simulink model "UorbRead"  (R2026a)
settings: Solver=FixedStepAuto  StopTime=inf  EnableMultiTasking=on
libraries: px4Peripheralslib x1, px4uORBlib x1
settings Model: ExtModeTrigDuration=10  Creator=Carlos Fabian  LastModifiedBy=Carlos Fabian
settings SolverCC: PositivePriorityOrder=on
settings HardwareCC: ProdLargestAtomicInteger=Long  ProdLargestAtomicFloat=Double  ProdHWDeviceType=ARM Compatible->ARM Cortex
settings SFSimCC: SimTargetLang=C++
settings RTWCC: SystemTargetFile=ert.tlc  HardwareBoard=PX4 Host Target  TLCOptions="-aInlineSetEventsForThisBaseRateFcn=TLC_FALSE -aSuppressMultiTaskScheduler=TLC_FALSE  -aRateBasedStepFcn=0"  Toolchain=GNU Tools for PX4 Autopilots  PortableWordSizes=on  TargetLang=C++  Description=Embedded Coder
settings ERTTargetCC: ExtModeTransport=2.0

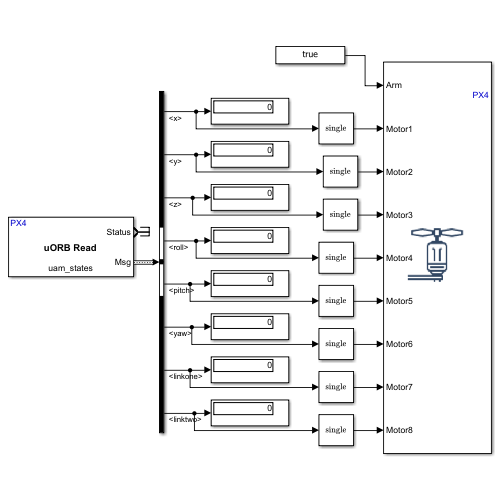
[thumbnail: Simulink's stored preview of the top-level diagram]
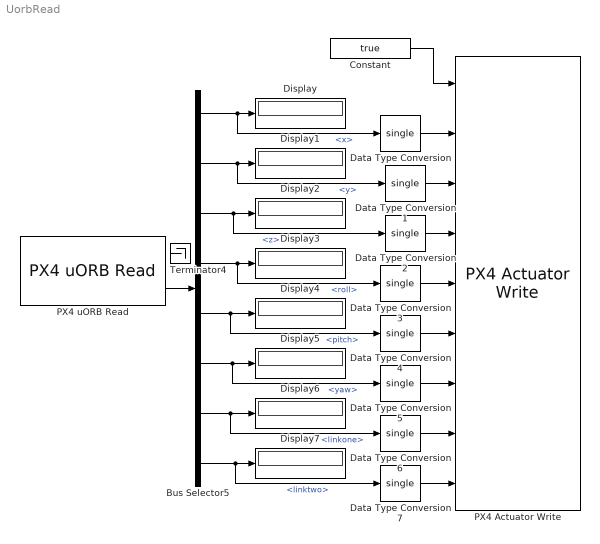
== system UorbRead ==
  Bus Selector5 : BusSelector  OutputSignals=x,y,z,roll,pitch,yaw,linkone,linktwo
  Constant : Constant  Value=true  SampleTime=0.01
  Data Type Conversion{,1..7} (8 alike) : DataTypeConversion  OutDataTypeStr=single  SaturateOnIntegerOverflow=off  RndMeth=Floor
  Display{,1..7} (8 alike) : Display
  PX4 Actuator Write : px4Peripheralslib/PX4 Actuator Write  Motor1Enable=on  Motor2Enable=on  Motor3Enable=on  Motor4Enable=on  Motor5Enable=on  Motor6Enable=on  Motor7Enable=on  Motor8Enable=on  Motor9Enable=off  Motor10Enable=off  Motor11Enable=off  Motor12Enable=off  IsMotorArray=off  Servo1Enable=off  Servo2Enable=off  Servo3Enable=off  Servo4Enable=off  Servo5Enable=off  Servo6Enable=off  Servo7Enable=off  Servo8Enable=off  IsServoArray=off
  PX4 uORB Read : px4uORBlib/PX4 uORB Read  uORBMsg=UamStates  uORBTopicName=uam_states  SubscribeNonZeroInstance=off  selectInstanceNum=1  SampleTime=0.01  isSingleTopicMsg=on  BlockingMode=off  BlockTimeout=1e-3
  Terminator4 : Terminator
  wires:
  PX4 uORB Read/2 -> Bus Selector5/1
  Bus Selector5/1 -> Data Type Conversion/1, Display/1  "<x>"
  Bus Selector5/2 -> Data Type Conversion1/1, Display1/1  "<y>"
  Bus Selector5/3 -> Data Type Conversion2/1, Display2/1  "<z>"
  Bus Selector5/4 -> Data Type Conversion3/1, Display3/1  "<roll>"
  Bus Selector5/5 -> Data Type Conversion4/1, Display4/1  "<pitch>"
  Bus Selector5/6 -> Data Type Conversion5/1, Display5/1  "<yaw>"
  Bus Selector5/7 -> Data Type Conversion6/1, Display6/1  "<linkone>"
  Bus Selector5/8 -> Data Type Conversion7/1, Display7/1  "<linktwo>"
  Constant/1 -> PX4 Actuator Write/1
  Data Type Conversion/1 -> PX4 Actuator Write/2
  Data Type Conversion1/1 -> PX4 Actuator Write/3
  Data Type Conversion2/1 -> PX4 Actuator Write/4
  Data Type Conversion3/1 -> PX4 Actuator Write/5
  Data Type Conversion4/1 -> PX4 Actuator Write/6
  Data Type Conversion5/1 -> PX4 Actuator Write/7
  Data Type Conversion6/1 -> PX4 Actuator Write/8
  Data Type Conversion7/1 -> PX4 Actuator Write/9
